simulink model "INS"  (R2018b)
settings: configuration reference "ins_config" (kept outside this file)
values from neighbouring files (symbols this model uses):
  INS_EXPORT = Simulink.Parameter(INS_EXPORT_VALUE)    [ins_model_init.m]
  INS_PARAM = Simulink.Parameter(INS_PARAM_VALUE)    [ins_model_init.m]
undefined symbols (not defined in the file or in its folder): DiscIntNeverNeededParam, INS_CONST, INS_EXPORT_VALUE, Sensor_Meas
libraries: simulink x131, FMT_Model_Lib x48
(part 1 of 6)
settings Model: SimulationMode=accelerator  Creator=jc  LastModifiedBy=zouji
settings ConfigSetRef: SourceLocation=Base Workspace

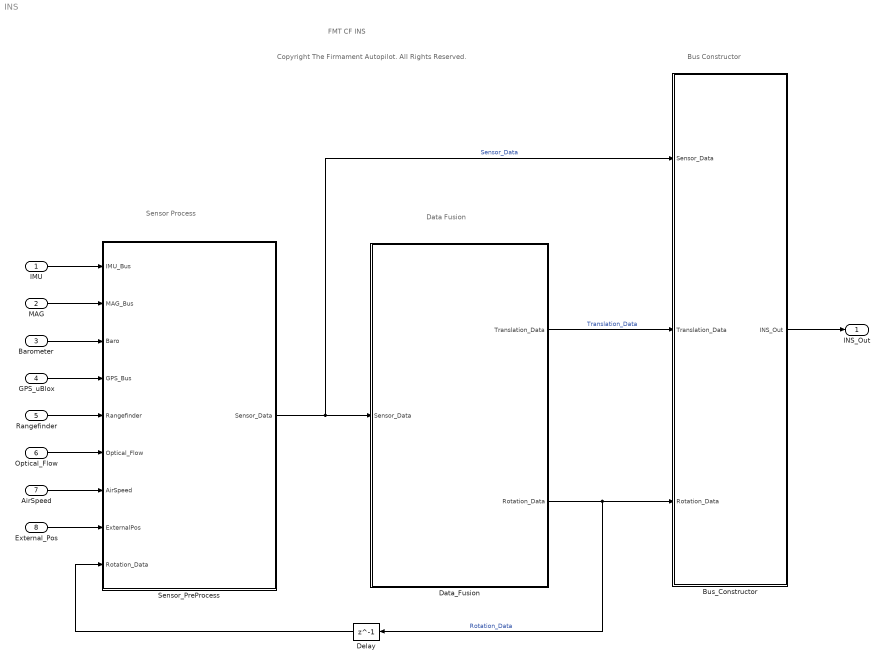
== system INS ==
  note: FMT CF INS
  note: Sensor Process
  note: Data Fusion
  note: Bus Constructor
  note: Copyright The Firmament Autopilot. All Rights Reserved.
  IMU : Inport  OutDataTypeStr=Bus: IMU_Bus  PortDimensions=[1 1]  SampleTime=[INS_CONST.dt,0]  Interpolate=off  BusOutputAsStruct=on
  MAG : Inport  Port=2  OutDataTypeStr=Bus: MAG_Bus  PortDimensions=[1 1]  SampleTime=[INS_CONST.dt,0]  Interpolate=off  BusOutputAsStruct=on
  Barometer : Inport  Port=3  OutDataTypeStr=Bus: Barometer_Bus  PortDimensions=[1 1]  SampleTime=[INS_CONST.dt,0]  Interpolate=off  BusOutputAsStruct=on
  GPS_uBlox : Inport  Port=4  OutDataTypeStr=Bus: GPS_uBlox_Bus  PortDimensions=[1 1]  SampleTime=[INS_CONST.dt,0]  Interpolate=off  BusOutputAsStruct=on
  Rangefinder : Inport  Port=5  OutDataTypeStr=Bus: Rangefinder_Bus  PortDimensions=1  SampleTime=[INS_CONST.dt,0]  Interpolate=off  BusOutputAsStruct=on
  Optical_Flow : Inport  Port=6  OutDataTypeStr=Bus: Optical_Flow_Bus  PortDimensions=[1 1]  SampleTime=[INS_CONST.dt,0]  Interpolate=off  BusOutputAsStruct=on
  AirSpeed : Inport  Port=7  OutDataTypeStr=Bus: AirSpeed_Bus  PortDimensions=[1 1]  SampleTime=[INS_CONST.dt,0]  Interpolate=off  BusOutputAsStruct=on
  External_Pos : Inport  Port=8  OutDataTypeStr=Bus: External_Pos_Bus  PortDimensions=[1 1]  SampleTime=[INS_CONST.dt,0]  Interpolate=off  BusOutputAsStruct=on
  Bus_Constructor : Subsystem  TreatAsAtomicUnit=on
  Data_Fusion : Subsystem  TreatAsAtomicUnit=on
  Delay : Delay  DelayLength=1
  Sensor_PreProcess : Subsystem  TreatAsAtomicUnit=on
  INS_Out : Outport  OutDataTypeStr=Bus: INS_Out_Bus
  wires:
  IMU/1 -> Sensor_PreProcess/1(IMU_Bus)
  MAG/1 -> Sensor_PreProcess/2(MAG_Bus)
  Barometer/1 -> Sensor_PreProcess/3(Baro)
  GPS_uBlox/1 -> Sensor_PreProcess/4(GPS_Bus)
  Rangefinder/1 -> Sensor_PreProcess/5(Rangefinder)
  Bus_Constructor/1(INS_Out) -> INS_Out/1
  Sensor_PreProcess/1(Sensor_Data) -> Bus_Constructor/1(Sensor_Data), Data_Fusion/1(Sensor_Data)  "Sensor_Data"
  Data_Fusion/2(Rotation_Data) -> Delay/1, Bus_Constructor/3(Rotation_Data)  "Rotation_Data"
  Data_Fusion/1(Translation_Data) -> Bus_Constructor/2(Translation_Data)  "Translation_Data"
  Delay/1 -> Sensor_PreProcess/9(Rotation_Data)
  Optical_Flow/1 -> Sensor_PreProcess/6(Optical_Flow)
  AirSpeed/1 -> Sensor_PreProcess/7(AirSpeed)
  External_Pos/1 -> Sensor_PreProcess/8(ExternalPos)

== system INS/Bus_Constructor ==
  Sensor_Data : Inport
  Translation_Data : Inport  Port=2
  Rotation_Data : Inport  Port=3
  Bus Creator : BusCreator  Inputs=29  OutDataTypeStr=Bus: INS_Out_Bus
      settings: InheritFromInputs=off
  Counter : Subsystem  TreatAsAtomicUnit=on
  Rotation_Output : Subsystem  TreatAsAtomicUnit=on
  Status_Output : Subsystem  TreatAsAtomicUnit=on
  Translation_Output : Subsystem  TreatAsAtomicUnit=on
  INS_Out : Outport  OutDataTypeStr=Bus: INS_Out_Bus
  wires:
  Bus Creator/1 -> INS_Out/1
  Counter/1(timestamp_ms) -> Bus Creator/1  "timestamp"
  Rotation_Output/2(theta) -> Bus Creator/3  "theta"
  Rotation_Output/1(phi) -> Bus Creator/2  "phi"
  Rotation_Output/4(att_quat) -> Bus Creator/5  "quat"
  Rotation_Output/3(psi) -> Bus Creator/4  "psi"
  Rotation_Output/5(p) -> Bus Creator/6  "p"
  Rotation_Output/6(q) -> Bus Creator/7  "q"
  Rotation_Output/7(r) -> Bus Creator/8  "r"
  Rotation_Output/8(ax) -> Bus Creator/9  "ax"
  Rotation_Output/9(ay) -> Bus Creator/10  "ay"
  Rotation_Output/10(az) -> Bus Creator/11  "az"
  Translation_Output/1(velN) -> Bus Creator/12  "vn"
  Translation_Output/2(velE) -> Bus Creator/13  "ve"
  Translation_Output/3(velD) -> Bus Creator/14  "vd"
  Status_Output/1(flags) -> Bus Creator/28  "flag"
  Status_Output/2(status) -> Bus Creator/29  "status"
  Translation_Output/13(x_R_m) -> Bus Creator/24  "x_R"
  Translation_Output/14(y_R_m) -> Bus Creator/25  "y_R"
  Translation_Output/15(h_R_m) -> Bus Creator/26  "h_R"
  Translation_Output/16(h_AGL_m) -> Bus Creator/27  "h_AGL"
  Translation_Data/1 -> Status_Output/1(Translation_Data), Translation_Output/1(Translation_Data), Rotation_Output/2(Translation_Data)
  Rotation_Data/1 -> Status_Output/2(Rotation_Data), Rotation_Output/1(Rotation_Data)
  Sensor_Data/1 -> Status_Output/3(Sensor_Data)
  Translation_Output/5(latitude) -> Bus Creator/16  "lat"
  Translation_Output/6(longitude) -> Bus Creator/17  "lon"
  Translation_Output/7(altitude) -> Bus Creator/18  "alt"
  Translation_Output/8(latitude_0) -> Bus Creator/19  "lat_0"
  Translation_Output/9(lontitude_0) -> Bus Creator/20  "lon_0"
  Translation_Output/10(altitude_0) -> Bus Creator/21  "alt_0"
  Translation_Output/4(airspeed) -> Bus Creator/15  "airspeed"
  Translation_Output/11(dx_dlat) -> Bus Creator/22  "dx_dlat"
  Translation_Output/12(dy_dlon) -> Bus Creator/23  "dy_dlon"

== system INS/Data_Fusion ==
  Sensor_Data : Inport
  Delay : Delay  DelayLength=1
  Rotation_Filter : Subsystem
  Translation_Filter : Subsystem
  Translation_Data : Outport
  Rotation_Data : Outport  Port=2
  wires:
  Rotation_Filter/1(Rotation_Data) -> Translation_Filter/2(Rotation_Data), Rotation_Data/1
  Translation_Filter/1(Translation_Data) -> Delay/1, Translation_Data/1
  Sensor_Data/1 -> Rotation_Filter/1(Sensor_Data), Translation_Filter/1(Sensor_Data)
  Delay/1 -> Rotation_Filter/2(Translation_Data)

== system INS/Sensor_PreProcess ==
  IMU_Bus : Inport  Interpolate=off  BusOutputAsStruct=on
  MAG_Bus : Inport  Port=2  Interpolate=off  BusOutputAsStruct=on
  Baro : Inport  Port=3  Interpolate=off  BusOutputAsStruct=on
  GPS_Bus : Inport  Port=4  Interpolate=off  BusOutputAsStruct=on
  Rangefinder : Inport  Port=5
  Optical_Flow : Inport  Port=6
  AirSpeed : Inport  Port=7
  ExternalPos : Inport  Port=8
  Rotation_Data : Inport  Port=9
  AirSpeed_Process : Subsystem  TreatAsAtomicUnit=on
  Baro_PreProcess : Subsystem  TreatAsAtomicUnit=on
  Bus Creator : BusCreator  Inputs=8
  ExternalPos_Process : Subsystem  TreatAsAtomicUnit=on
  GPS_PreProcess : Subsystem  TreatAsAtomicUnit=on
  IMU_PreProcess : Subsystem  TreatAsAtomicUnit=on
  MAG_PreProcess : Subsystem  TreatAsAtomicUnit=on
  OpticalFlow_PreProcess : Subsystem  TreatAsAtomicUnit=on
  Rangefinder_PreProcess : Subsystem  TreatAsAtomicUnit=on
  Sensor_Data : Outport
  wires:
  IMU_Bus/1 -> OpticalFlow_PreProcess/2(IMU_Data), IMU_PreProcess/1(IMU_Bus)
  GPS_Bus/1 -> GPS_PreProcess/1(GPS_Bus)
  GPS_PreProcess/1(GPS_Data) -> MAG_PreProcess/3(GPS_Data), Bus Creator/3  "GPS_Data"
  MAG_Bus/1 -> MAG_PreProcess/1(MAG_Bus)
  Rotation_Data/1 -> Rangefinder_PreProcess/1(Rotation_Data), MAG_PreProcess/2(Rotation_Data)
  Baro/1 -> Baro_PreProcess/1(Baro)
  IMU_PreProcess/1(IMU_Data) -> Bus Creator/1  "IMU_Data"
  MAG_PreProcess/1(Mag_Data) -> Bus Creator/2  "Mag_Data"
  Baro_PreProcess/1(Baro_Data) -> Bus Creator/4  "Baro_Data"
  Bus Creator/1 -> Sensor_Data/1
  Rangefinder/1 -> Rangefinder_PreProcess/2(Rangefinder_Bus)
  Rangefinder_PreProcess/1(Rangefinder_Data) -> OpticalFlow_PreProcess/1(Rangefinder_Data), Bus Creator/5  "Rangefinder_Data"
  OpticalFlow_PreProcess/1(OpticalFlow_Data) -> Bus Creator/6  "OpticalFlow_Data"
  Optical_Flow/1 -> OpticalFlow_PreProcess/3(OpticalFlow_Bus)
  AirSpeed_Process/1(AirSpeed_Data) -> Bus Creator/7  "AirSpeed_Data"
  AirSpeed/1 -> AirSpeed_Process/1(AirSpeed)
  ExternalPos/1 -> ExternalPos_Process/1(ExternalPos)
  ExternalPos_Process/1(ExternalPos_Data) -> Bus Creator/8  "ExternalPos_Data"

== system INS/Bus_Constructor/Counter ==
  Add : Sum
  Constant : Constant  Value=INS_EXPORT.period  OutDataTypeStr=uint32
  Data Type Conversion : DataTypeConversion  OutDataTypeStr=uint32
  Output : UnitDelay  InitialCondition=0.0  SampleTime=-1
  timestamp_ms : Outport
  wires:
  Add/1 -> Output/1
  Output/1 -> Add/2, Data Type Conversion/1
  Data Type Conversion/1 -> timestamp_ms/1
  Constant/1 -> Add/1

== system INS/Bus_Constructor/Rotation_Output ==
  Rotation_Data : Inport
  Translation_Data : Inport  Port=2
  Bus Selector : BusSelector  OutputSignals=ba_mPs2
  Bus Selector3 : BusSelector  OutputSignals=phi_rad,theta_rad,psi_rad,att_quat,gyr_B_radPs,acc_B_mPs2,M_BO
  Demux3 : Demux  Outputs=3
  Demux4 : Demux  Outputs=3
  Multiply : Product  Multiplication=Matrix(*)
  Signal Copy : SignalConversion  OverrideOpt=off
  Sum : Sum  Inputs=|+-
  phi : Outport
  theta : Outport  Port=2
  psi : Outport  Port=3
  att_quat : Outport  Port=4
  p : Outport  Port=5
  q : Outport  Port=6
  r : Outport  Port=7
  ax : Outport  Port=8
  ay : Outport  Port=9
  az : Outport  Port=10
  wires:
  Bus Selector/1 -> Multiply/2  "<ba_mPs2>"
  Demux4/1 -> ax/1  "acc_x"
  Demux3/3 -> r/1  "gyr_z"
  Demux3/2 -> q/1  "gyr_y"
  Demux3/1 -> p/1  "gyr_x"
  Bus Selector3/5 -> Demux3/1  "<gyr_B_radPs>"
  Sum/1 -> Demux4/1
  Bus Selector3/1 -> phi/1  "<phi_rad>"
  Bus Selector3/6 -> Sum/1  "<acc_B_mPs2>"
  Demux4/3 -> az/1  "acc_z"
  Demux4/2 -> ay/1  "acc_y"
  Bus Selector3/2 -> theta/1  "<theta_rad>"
  Bus Selector3/3 -> psi/1  "<psi_rad>"
  Bus Selector3/7 -> Multiply/1  "<M_BO>"
  Multiply/1 -> Sum/2
  Bus Selector3/4 -> att_quat/1  "<att_quat>"
  Rotation_Data/1 -> Signal Copy/1
  Signal Copy/1 -> Bus Selector3/1
  Translation_Data/1 -> Bus Selector/1

== system INS/Bus_Constructor/Status_Output ==
  Translation_Data : Inport
  Rotation_Data : Inport  Port=2
  Sensor_Data : Inport  Port=3
  INS_Flag : Subsystem
  INS_Quality : Subsystem
  Sensor_Status : Subsystem
  flags : Outport
  status : Outport  Port=2
  wires:
  INS_Flag/1(flags) -> flags/1
  Sensor_Status/1(status) -> status/1
  INS_Quality/1(ins_valid) -> INS_Flag/1(INS_Valid)
  Rotation_Data/1 -> INS_Flag/3(Rotation_Data)
  Sensor_Data/1 -> Sensor_Status/1(Sensor_Data), INS_Flag/2(Sensor_Data), INS_Quality/2(Sensor_Data)
  Translation_Data/1 -> INS_Quality/1(Translation_Data)

== system INS/Bus_Constructor/Translation_Output ==
  Translation_Data : Inport
  Bus Selector4 : BusSelector  OutputSignals=vn_mPs,ve_mPs,vd_mPs,TAS_mPs,lat_rad,lon_rad,h_m,lat_0_rad,lon_0_rad,h_0_m,dx_dlat,dy_dlon,x_R_m,y_R_m,h_R_m,h_gnd_m
  Signal Copy : SignalConversion  OverrideOpt=off
  velN : Outport
  velE : Outport  Port=2
  velD : Outport  Port=3
  airspeed : Outport  Port=4
  latitude : Outport  Port=5
  longitude : Outport  Port=6
  altitude : Outport  Port=7
  latitude_0 : Outport  Port=8
  lontitude_0 : Outport  Port=9
  altitude_0 : Outport  Port=10
  dx_dlat : Outport  Port=11
  dy_dlon : Outport  Port=12
  x_R_m : Outport  Port=13
  y_R_m : Outport  Port=14
  h_R_m : Outport  Port=15
  h_AGL_m : Outport  Port=16
  wires:
  Bus Selector4/5 -> latitude/1  "<lat_rad>"
  Bus Selector4/6 -> longitude/1  "<lon_rad>"
  Bus Selector4/2 -> velE/1  "<ve_mPs>"
  Bus Selector4/3 -> velD/1  "<vd_mPs>"
  Bus Selector4/7 -> altitude/1  "<h_m>"
  Bus Selector4/1 -> velN/1  "<vn_mPs>"
  Bus Selector4/16 -> h_AGL_m/1  "<h_gnd_m>"
  Bus Selector4/15 -> h_R_m/1  "<h_R_m>"
  Bus Selector4/13 -> x_R_m/1  "<x_R_m>"
  Bus Selector4/14 -> y_R_m/1  "<y_R_m>"
  Translation_Data/1 -> Signal Copy/1
  Bus Selector4/8 -> latitude_0/1  "<lat_0_rad>"
  Bus Selector4/9 -> lontitude_0/1  "<lon_0_rad>"
  Bus Selector4/10 -> altitude_0/1  "<h_0_m>"
  Bus Selector4/11 -> dx_dlat/1  "<dx_dlat>"
  Bus Selector4/12 -> dy_dlon/1  "<dy_dlon>"
  Signal Copy/1 -> Bus Selector4/1
  Bus Selector4/4 -> airspeed/1  "<TAS_mPs>"

== system INS/Data_Fusion/Rotation_Filter ==
  Sensor_Data : Inport
  Translation_Data : Inport  Port=2
  AHRS : Subsystem  TreatAsAtomicUnit=on
  RF_Data_PreProcess : Subsystem  TreatAsAtomicUnit=on
  Rotation_Data : Outport
  wires:
  Sensor_Data/1 -> AHRS/2(Sensor_Data), RF_Data_PreProcess/1(Sensor_Data)
  AHRS/1(Rotation_Data) -> Rotation_Data/1
  RF_Data_PreProcess/1(RF_Data) -> AHRS/1(RF_Data)  "RF_Data"
  Translation_Data/1 -> AHRS/3(Translation_Data)

== system INS/Data_Fusion/Translation_Filter ==
  Sensor_Data : Inport
  Rotation_Data : Inport  Port=2
  CF : Subsystem  TreatAsAtomicUnit=on
  Delay : Delay  DelayLength=1
  TF_Data_PreProcess : Subsystem  TreatAsAtomicUnit=on
  Translation_Data : Outport
  wires:
  CF/1(Translation_Data) -> Delay/1, Translation_Data/1
  TF_Data_PreProcess/1(TF_Data) -> CF/1(TF_Data)  "TF_Data"
  Sensor_Data/1 -> TF_Data_PreProcess/1(Sensor_Data)
  Delay/1 -> TF_Data_PreProcess/3(Translation_Data)
  Rotation_Data/1 -> TF_Data_PreProcess/2(Rotation_Data), CF/2(Rotation_Data)

== system INS/Sensor_PreProcess/AirSpeed_Process ==
  AirSpeed : Inport
  Bus Creator : BusCreator  Inputs=3
  Bus Selector : BusSelector  OutputSignals=timestamp,diff_pressure
  Calculate_IAS : Subsystem
  Saturation1 : Saturate  UpperLimit=999  LowerLimit=0.1
  Sensor_Valid : Subsystem  mask{max_pressure=1e4, min_pressure=-1e4, max_temp=80, min_temp=-20, timeout=200}
      mask prompts: max_pressure "Max pressure (Pa)"; min_pressure "Min pressure (Pa)"; max_temp "Max temprature (deg)"; min_temp "Min temprature (deg)"; timeout "Timeout (ms)"
  AirSpeed_Data : Outport
  wires:
  Bus Creator/1 -> AirSpeed_Data/1
  AirSpeed/1 -> Bus Selector/1, Sensor_Valid/1(Airspeed)
  Bus Selector/1 -> Bus Creator/1  "<timestamp>"
  Bus Selector/2 -> Calculate_IAS/1(diff_pressure)  "<diff_pressure>"
  Calculate_IAS/1(IAS) -> Saturation1/1
  Saturation1/1 -> Bus Creator/2  "IAS"
  Sensor_Valid/1(valid) -> Bus Creator/3  "valid"

== system INS/Sensor_PreProcess/Baro_PreProcess ==
  Baro : Inport
  Bus Creator : BusCreator  Inputs=5
  Bus Selector1 : BusSelector  OutputSignals=pressure
  Bus Selector2 : BusSelector  OutputSignals=temperature,timestamp
  Pressure_Height : Subsystem
  Relative_Height : Subsystem
  Sensor_Valid : Subsystem  mask{max_pressure=110e3, min_pressure=30e3, max_temp=70, min_temp=-20, timeout=200}
      mask prompts: max_pressure "Max pressure (Pa)"; min_pressure "Min pressure (Pa)"; max_temp "Max temprature (deg)"; min_temp "Min temprature (deg)"; timeout "Timeout (ms)"
  Baro_Data : Outport
  wires:
  Bus Selector1/1 -> Pressure_Height/1(pressure_Pa)  "<pressure>"
  Baro/1 -> Bus Selector2/1, Bus Selector1/1, Sensor_Valid/1(Baro), Relative_Height/1(Baro)
  Bus Creator/1 -> Baro_Data/1
  Bus Selector2/1 -> Bus Creator/4  "<temperature>"
  Bus Selector2/2 -> Bus Creator/5  "<timestamp>"
  Pressure_Height/1(h_FL_m) -> Relative_Height/3(h_FL_m), Bus Creator/3  "h_FL_m"
  Sensor_Valid/1(valid) -> Relative_Height/2(data_valid)
  Relative_Height/2(baro_valid) -> Bus Creator/2  "baro_valid"
  Relative_Height/1(h_R_m) -> Bus Creator/1  "h_R_m"

== system INS/Sensor_PreProcess/ExternalPos_Process ==
  ExternalPos : Inport
  Bus Creator : BusCreator  Inputs=11
  Bus Selector : BusSelector  OutputSignals=timestamp,field_valid
  Bus_Selector : Subsystem
  Sensor_Valid : Subsystem  mask{timeout=200}
      mask prompts: timeout "Timeout (ms)"
  Signal Copy : SignalConversion  OverrideOpt=off
  ExternalPos_Data : Outport
  wires:
  Bus Creator/1 -> ExternalPos_Data/1
  ExternalPos/1 -> Bus_Selector/1(ExternalPos), Bus Selector/1
  Bus Selector/1 -> Signal Copy/1, Sensor_Valid/1(timestamp)  "<timestamp>"
  Signal Copy/1 -> Bus Creator/1  "timestamp"
  Sensor_Valid/1(pos_valid) -> Bus Creator/2  "pos_valid"
  Sensor_Valid/2(height_valid) -> Bus Creator/3  "height_valid"
  Sensor_Valid/3(att_valid) -> Bus Creator/4  "att_valid"
  Sensor_Valid/4(heading_valid) -> Bus Creator/5  "heading_valid"
  Bus_Selector/1(x) -> Bus Creator/6  "x"
  Bus_Selector/2(y) -> Bus Creator/7  "y"
  Bus_Selector/3(h) -> Bus Creator/8  "h"
  Bus_Selector/4(phi) -> Bus Creator/9  "phi"
  Bus_Selector/5(theta) -> Bus Creator/10  "theta"
  Bus_Selector/6(psi) -> Bus Creator/11  "psi"
  Bus Selector/2 -> Sensor_Valid/2(field_valid)  "<field_valid>"

== system INS/Sensor_PreProcess/GPS_PreProcess ==
  GPS_Bus : Inport  Interpolate=off  BusOutputAsStruct=on
  Bus Creator1 : BusCreator  Inputs=20
  Compare To Constant : simulink/Logic and Bit Operations/Compare To Constant  relop=>  const=0  OutDataTypeStr=boolean
  Compare To Constant1 : simulink/Logic and Bit Operations/Compare To Constant  relop===  const=2  OutDataTypeStr=boolean
  Data_Scalling : Subsystem
  Status_Quality : Subsystem
  WGS84_Model : Subsystem
  GPS_Data : Outport
  wires:
  Compare To Constant1/1 -> Bus Creator1/1  "GPS_valid"
  WGS84_Model/5(dz_dh) -> Bus Creator1/10  "dz_dh"
  GPS_Bus/1 -> Data_Scalling/1(GPS_Bus), Status_Quality/1(GPS_Bus)
  Compare To Constant/1 -> WGS84_Model/Trigger
  Bus Creator1/1 -> GPS_Data/1
  Status_Quality/1(gps_status) -> Compare To Constant/1, Compare To Constant1/1
  WGS84_Model/2(lat_0_rad) -> Bus Creator1/7  "lat_0_rad"
  WGS84_Model/3(dx_dlat) -> Bus Creator1/8  "dx_dlat"
  WGS84_Model/4(dy_dlon) -> Bus Creator1/9  "dy_dlon"
  Status_Quality/2(spd_quality) -> Bus Creator1/2  "spd_quality"
  Status_Quality/3(hor_pos_quality) -> Bus Creator1/3  "pos_quality"
  Data_Scalling/2(lon_O_rad) -> WGS84_Model/2(lon_rad), Bus Creator1/12  "lon_rad"
  Data_Scalling/3(height_O_m) -> WGS84_Model/3(alt_m), Bus Creator1/13  "height_m"
  Data_Scalling/1(lat_O_rad) -> Bus Creator1/11, WGS84_Model/1(lat_rad)  "lat_rad"
  Data_Scalling/4(vn_O_mPs) -> Bus Creator1/14  "vn_mPs"
  Data_Scalling/5(ve_O_mPs) -> Bus Creator1/15  "ve_mPs"
  Data_Scalling/6(vd_O_mPs) -> Bus Creator1/16  "vd_mPs"
  Data_Scalling/8(numSV) -> Bus Creator1/18  "numSV"
  Data_Scalling/10(timestamp_ms) -> Bus Creator1/20  "timestamp_ms"
  WGS84_Model/1(lon_0_rad) -> Bus Creator1/6  "lon_0_rad"
  Status_Quality/4(ver_pos_quality) -> Bus Creator1/4  "alt_quality"
  Data_Scalling/9(fixType) -> Bus Creator1/19  "fixType"
  Data_Scalling/7(heading_rad) -> Bus Creator1/17  "heading_rad"
  Status_Quality/5(heading_valid) -> Bus Creator1/5  "heading_valid"

== system INS/Sensor_PreProcess/IMU_PreProcess ==
  IMU_Bus : Inport
  Bus Creator : BusCreator  Inputs=3
  Data_Select : Subsystem
  Sensor_Valid : Subsystem  mask{gyr_min=-2200*pi/180, gyr_max=2200*pi/180, acc_min=-10*INS_CONST.g, acc_max=10*INS_CONST.g, timeout=100}
      mask prompts: gyr_min "Gyro min (rad/s)"; gyr_max "Gyro max (rad/s)"; acc_min "Accel min (m/s2)"; acc_max "Accel max (m/s2)"; timeout "Timeout (ms)"
  IMU_Data : Outport
  wires:
  Bus Creator/1 -> IMU_Data/1
  Sensor_Valid/1(valid) -> Bus Creator/3  "IMU_valid"
  Data_Select/3(timestamp_ms) -> Sensor_Valid/3(timestamp_ms)
  Data_Select/2(acc_B_mPs2) -> Bus Creator/2, Sensor_Valid/2(acc_B_mPs2)  "acc_B_mPs2"
  Data_Select/1(gyr_B_radPs) -> Bus Creator/1, Sensor_Valid/1(gyr_B_radPs)  "gyr_B_radPs"
  IMU_Bus/1 -> Data_Select/1(IMU_Bus)

== system INS/Sensor_PreProcess/MAG_PreProcess ==
  MAG_Bus : Inport
  Rotation_Data : Inport  Port=2
  GPS_Data : Inport  Port=3
  Bus Creator : BusCreator  Inputs=3
  Bus Selector4 : BusSelector  OutputSignals=M_OB
  Bus_Select : Subsystem
  Gauss_to_uT : Gain  Gain=100
  Mag_Data_Process : Subsystem
  Sensor_Valid : Subsystem  mask{mag_min=-30000, mag_max=30000, timeout=1000}
      mask prompts: mag_min "Mag min (gauss)"; mag_max "Mag max (gauss)"; timeout "Timeout (ms)"
  Mag_Data : Outport
  wires:
  Rotation_Data/1 -> Bus Selector4/1
  Bus Selector4/1 -> Mag_Data_Process/3(DCM_OB)  "<M_OB>"
  Gauss_to_uT/1 -> Mag_Data_Process/1(mag_B_uT)
  MAG_Bus/1 -> Bus_Select/1(MAG_Bus)
  Mag_Data_Process/1(mag_normalized_B) -> Bus Creator/1  "mag_norm_B"
  GPS_Data/1 -> Mag_Data_Process/4(GPS_Data)
  Mag_Data_Process/2(mag_quality) -> Bus Creator/2  "mag_quality"
  Bus Creator/1 -> Mag_Data/1
  Bus_Select/1(mag_B_gauss) -> Gauss_to_uT/1, Sensor_Valid/1(mag_B_gauss)
  Bus_Select/2(timestamp_ms) -> Sensor_Valid/2(timestamp_ms)
  Sensor_Valid/1(valid) -> Bus Creator/3, Mag_Data_Process/2(mag_valid)  "mag_valid"

== system INS/Sensor_PreProcess/OpticalFlow_PreProcess ==
  Rangefinder_Data : Inport
  IMU_Data : Inport  Port=2
  OpticalFlow_Bus : Inport  Port=3
  Bus Creator : BusCreator  Inputs=4
  Bus Selector : BusSelector  OutputSignals=timestamp
  Height_Compensation : Subsystem
  Sensor_Valid : Subsystem  mask{max_vel=20, min_vel=-20, q_high=90, q_low=50, timeout=100}
      mask prompts: max_vel "Max Velocity (m/s)"; min_vel "Min Velocity (m/s)"; q_high "Quality Threshold High"; q_low "Quality Threshold Low"; timeout "Timeout (ms)"
  OpticalFlow_Data : Outport
  wires:
  Bus Creator/1 -> OpticalFlow_Data/1
  Sensor_Valid/1(valid) -> Bus Creator/2  "valid"
  OpticalFlow_Bus/1 -> Height_Compensation/1(OpticalFlow_Bus), Bus Selector/1, Sensor_Valid/1(OpticalFlow_Bus)
  Rangefinder_Data/1 -> Sensor_Valid/2(Rangefinder_Data), Height_Compensation/3(Rangefinder_Data)
  Height_Compensation/1(vx_B_mPs) -> Bus Creator/3  "vx"
  Height_Compensation/2(vy_B_mPs) -> Bus Creator/4  "vy"
  Bus Selector/1 -> Bus Creator/1  "<timestamp>"
  IMU_Data/1 -> Height_Compensation/2(IMU_Data)

== system INS/Sensor_PreProcess/Rangefinder_PreProcess ==
  Rotation_Data : Inport
  Rangefinder_Bus : Inport  Port=2
  Bus Creator : BusCreator  Inputs=4
  Bus Selector : BusSelector  OutputSignals=timestamp
  Sensor_Valid : Subsystem  mask{max_alt=4, min_alt=0, timeout=100}
      mask prompts: max_alt "Max Altitude (m)"; min_alt "Min Altitude (m)"; timeout "Timeout (ms)"
  Subsystem : Subsystem
  Tilt_Compensation : Subsystem
  Rangefinder_Data : Outport
  wires:
  Rangefinder_Bus/1 -> Bus Selector/1, Sensor_Valid/1(Rangefinder_Bus), Tilt_Compensation/1(Rangefinder_Bus)
  Sensor_Valid/1(valid) -> Subsystem/1(in)
  Bus Creator/1 -> Rangefinder_Data/1
  Rotation_Data/1 -> Tilt_Compensation/2(Rotation_Data)
  Tilt_Compensation/2(distance) -> Bus Creator/4  "distance"
  Tilt_Compensation/1(raw_distance) -> Bus Creator/3  "raw_distance"
  Bus Selector/1 -> Bus Creator/1  "<timestamp>"
  Subsystem/1(out) -> Bus Creator/2  "valid"

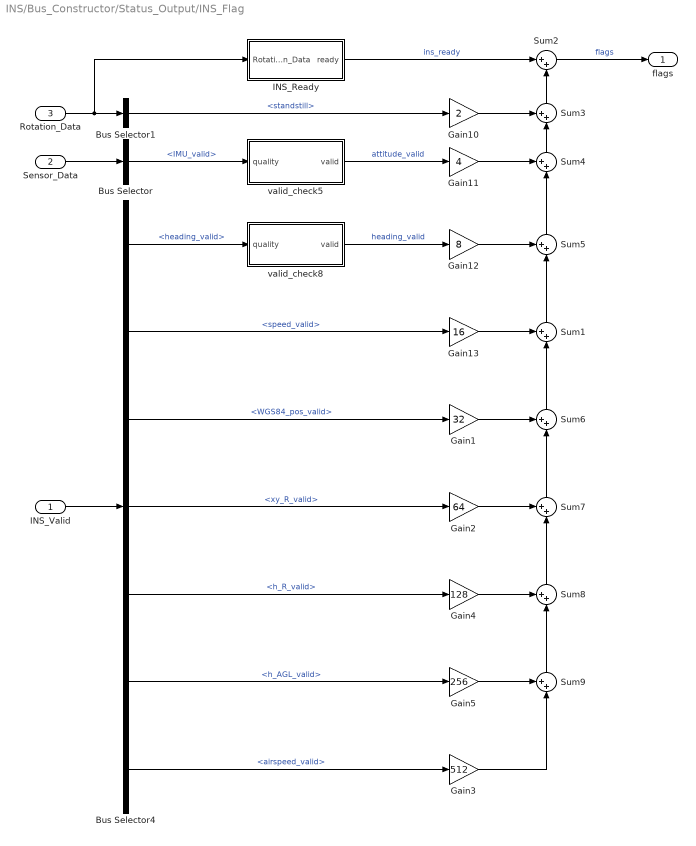
== system INS/Bus_Constructor/Status_Output/INS_Flag ==
  INS_Valid : Inport
  Sensor_Data : Inport  Port=2
  Rotation_Data : Inport  Port=3
  Bus Selector : BusSelector  OutputSignals=IMU_Data.IMU_valid
  Bus Selector1 : BusSelector  OutputSignals=standstill
  Bus Selector4 : BusSelector  OutputSignals=heading_valid,speed_valid,WGS84_pos_valid,xy_R_valid,h_R_valid,h_AGL_valid,airspeed_valid
  Gain1 : Gain  Gain=32  OutDataTypeStr=uint32
  Gain10 : Gain  Gain=2  OutDataTypeStr=uint32
  Gain11 : Gain  Gain=4  OutDataTypeStr=uint32
  Gain12 : Gain  Gain=8  OutDataTypeStr=uint32
  Gain13 : Gain  Gain=16  OutDataTypeStr=uint32
  Gain2 : Gain  Gain=64  OutDataTypeStr=uint32
  Gain3 : Gain  Gain=512  OutDataTypeStr=uint32
  Gain4 : Gain  Gain=128  OutDataTypeStr=uint32
  Gain5 : Gain  Gain=256  OutDataTypeStr=uint32
  INS_Ready : Subsystem
  Sum{1,3..9} (8 alike) : Sum  Inputs=++|
  Sum2 : Sum  Inputs=|++
  valid_check5 : Subsystem  mask{time_out=100}
      mask prompts: time_out "timeout in ms"
  valid_check8 : Subsystem  mask{time_out=1000}
      mask prompts: time_out "timeout in ms"
  flags : Outport
  wires:
  Bus Selector/1 -> valid_check5/1(quality)  "<IMU_valid>"
  Gain1/1 -> Sum6/1
  Sum1/1 -> Sum5/2
  Gain13/1 -> Sum1/1
  valid_check5/1(valid) -> Gain11/1  "attitude_valid"
  Bus Selector4/3 -> Gain1/1  "<WGS84_pos_valid>"
  Bus Selector4/2 -> Gain13/1  "<speed_valid>"
  Bus Selector4/1 -> valid_check8/1(quality)  "<heading_valid>"
  INS_Valid/1 -> Bus Selector4/1
  Sum2/1 -> flags/1  "flags"
  Sum5/1 -> Sum4/2
  INS_Ready/1(ready) -> Sum2/1  "ins_ready"
  Gain11/1 -> Sum4/1
  Gain12/1 -> Sum5/1
  Sum3/1 -> Sum2/2
  Sum4/1 -> Sum3/2
  Sensor_Data/1 -> Bus Selector/1
  Gain10/1 -> Sum3/1
  Sum6/1 -> Sum1/2
  Sum7/1 -> Sum6/2
  Rotation_Data/1 -> INS_Ready/1(Rotation_Data), Bus Selector1/1
  Gain2/1 -> Sum7/1
  Sum8/1 -> Sum7/2
  Gain4/1 -> Sum8/1
  Bus Selector4/4 -> Gain2/1  "<xy_R_valid>"
  Bus Selector4/5 -> Gain4/1  "<h_R_valid>"
  Bus Selector4/6 -> Gain5/1  "<h_AGL_valid>"
  valid_check8/1(valid) -> Gain12/1  "heading_valid"
  Bus Selector4/7 -> Gain3/1  "<airspeed_valid>"
  Sum9/1 -> Sum8/2
  Gain5/1 -> Sum9/1
  Gain3/1 -> Sum9/2
  Bus Selector1/1 -> Gain10/1  "<standstill>"

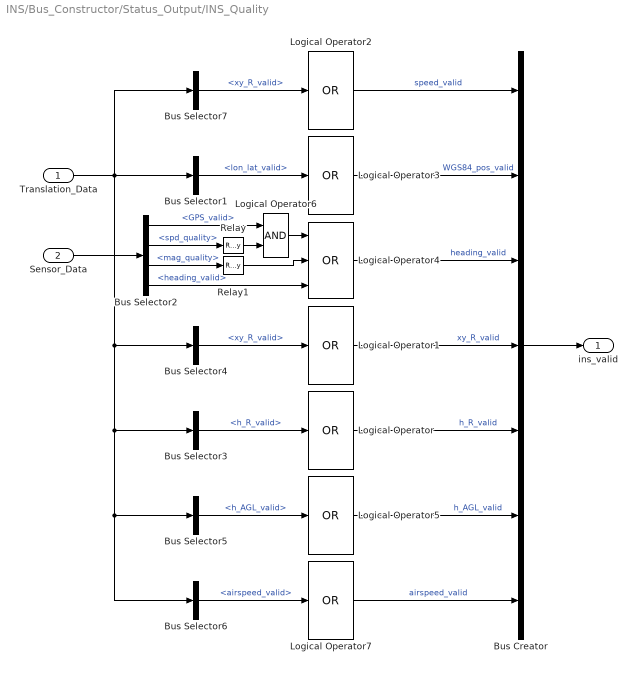
== system INS/Bus_Constructor/Status_Output/INS_Quality ==
  Translation_Data : Inport
  Sensor_Data : Inport  Port=2
  Bus Creator : BusCreator  Inputs=7
  Bus Selector1 : BusSelector  OutputSignals=sensor_valid.lon_lat_valid
  Bus Selector2 : BusSelector  OutputSignals=GPS_Data.GPS_valid,GPS_Data.spd_quality,Mag_Data.mag_quality,ExternalPos_Data.heading_valid
  Bus Selector3 : BusSelector  OutputSignals=sensor_valid.h_R_valid
  Bus Selector4 : BusSelector  OutputSignals=sensor_valid.xy_R_valid
  Bus Selector5 : BusSelector  OutputSignals=sensor_valid.h_AGL_valid
  Bus Selector6 : BusSelector  OutputSignals=sensor_valid.airspeed_valid
  Bus Selector7 : BusSelector  OutputSignals=sensor_valid.xy_R_valid
  Logical Operator{,1..3,5,7} (6 alike) : Logic  Operator=OR  Inputs=1  AllPortsSameDT=off  OutDataTypeStr=boolean
  Logical Operator4 : Logic  Operator=OR  Inputs=3  AllPortsSameDT=off  OutDataTypeStr=boolean
  Logical Operator6 : Logic  AllPortsSameDT=off  OutDataTypeStr=boolean
  Relay : Relay  OnSwitchValue=0.2  OffSwitchValue=0.1
  Relay1 : Relay  OnSwitchValue=0.3  OffSwitchValue=0.2  OutDataTypeStr=boolean
  ins_valid : Outport
  wires:
  Bus Creator/1 -> ins_valid/1
  Logical Operator4/1 -> Bus Creator/3  "heading_valid"
  Sensor_Data/1 -> Bus Selector2/1
  Bus Selector2/3 -> Relay1/1  "<mag_quality>"
  Bus Selector7/1 -> Logical Operator2/1  "<xy_R_valid>"
  Logical Operator3/1 -> Bus Creator/2  "WGS84_pos_valid"
  Logical Operator2/1 -> Bus Creator/1  "speed_valid"
  Logical Operator1/1 -> Bus Creator/4  "xy_R_valid"
  Logical Operator/1 -> Bus Creator/5  "h_R_valid"
  Bus Selector5/1 -> Logical Operator5/1  "<h_AGL_valid>"
  Translation_Data/1 -> Bus Selector6/1, Bus Selector5/1, Bus Selector3/1, Bus Selector4/1, Bus Selector1/1, Bus Selector7/1
  Relay1/1 -> Logical Operator4/2
  Bus Selector1/1 -> Logical Operator3/1  "<lon_lat_valid>"
  Bus Selector4/1 -> Logical Operator1/1  "<xy_R_valid>"
  Bus Selector3/1 -> Logical Operator/1  "<h_R_valid>"
  Logical Operator5/1 -> Bus Creator/6  "h_AGL_valid"
  Bus Selector2/2 -> Relay/1  "<spd_quality>"
  Bus Selector2/1 -> Logical Operator6/1  "<GPS_valid>"
  Relay/1 -> Logical Operator6/2
  Logical Operator6/1 -> Logical Operator4/1
  Bus Selector2/4 -> Logical Operator4/3  "<heading_valid>"
  Bus Selector6/1 -> Logical Operator7/1  "<airspeed_valid>"
  Logical Operator7/1 -> Bus Creator/7  "airspeed_valid"

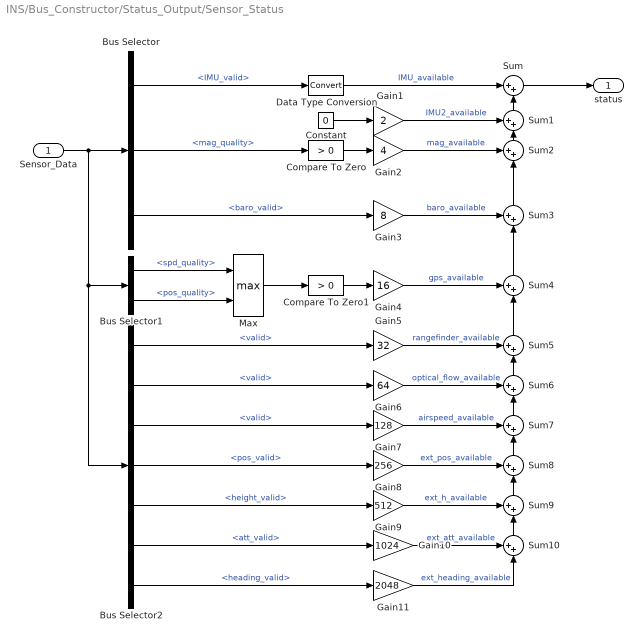
== system INS/Bus_Constructor/Status_Output/Sensor_Status ==
  Sensor_Data : Inport
  Bus Selector : BusSelector  OutputSignals=IMU_Data.IMU_valid,Mag_Data.mag_quality,Baro_Data.baro_valid
  Bus Selector1 : BusSelector  OutputSignals=GPS_Data.spd_quality,GPS_Data.pos_quality
  Bus Selector2 : BusSelector  OutputSignals=Rangefinder_Data.valid,OpticalFlow_Data.valid,AirSpeed_Data.valid,ExternalPos_Data.pos_valid,ExternalPos_Data.height_valid,ExternalPos_Data.att_valid,ExternalPos_Data.heading_valid
  Compare To Zero : simulink/Logic and Bit Operations/Compare To Zero  relop=>  OutDataTypeStr=boolean
  Compare To Zero1 : simulink/Logic and Bit Operations/Compare To Zero  relop=>  OutDataTypeStr=boolean
  Constant : Constant  Value=0  OutDataTypeStr=Inherit: Inherit via back propagation
  Data Type Conversion : DataTypeConversion
  Gain1 : Gain  Gain=2  OutDataTypeStr=uint32
  Gain10 : Gain  Gain=1024  OutDataTypeStr=uint32
  Gain11 : Gain  Gain=2048  OutDataTypeStr=uint32
  Gain2 : Gain  Gain=4  OutDataTypeStr=uint32
  Gain3 : Gain  Gain=8  OutDataTypeStr=uint32
  Gain4 : Gain  Gain=16  OutDataTypeStr=uint32
  Gain5 : Gain  Gain=32  OutDataTypeStr=uint32
  Gain6 : Gain  Gain=64  OutDataTypeStr=uint32
  Gain7 : Gain  Gain=128  OutDataTypeStr=uint32
  Gain8 : Gain  Gain=256  OutDataTypeStr=uint32
  Gain9 : Gain  Gain=512  OutDataTypeStr=uint32
  Max : MinMax  Function=max  Inputs=2
  Sum : Sum  Inputs=|++
  Sum{1..10} (10 alike) : Sum  Inputs=++|
  status : Outport
  wires:
  Max/1 -> Compare To Zero1/1
  Compare To Zero1/1 -> Gain4/1
  Bus Selector1/2 -> Max/2  "<pos_quality>"
  Bus Selector1/1 -> Max/1  "<spd_quality>"
  Sum4/1 -> Sum3/2
  Gain3/1 -> Sum3/1  "baro_available"
  Sum3/1 -> Sum2/2
  Gain2/1 -> Sum2/1  "mag_available"
  Compare To Zero/1 -> Gain2/1
  Sum2/1 -> Sum1/2
  Bus Selector/3 -> Gain3/1  "<baro_valid>"
  Bus Selector/2 -> Compare To Zero/1  "<mag_quality>"
  Sensor_Data/1 -> Bus Selector/1, Bus Selector2/1, Bus Selector1/1
  Sum/1 -> status/1
  Data Type Conversion/1 -> Sum/1  "IMU_available"
  Bus Selector/1 -> Data Type Conversion/1  "<IMU_valid>"
  Constant/1 -> Gain1/1
  Sum1/1 -> Sum/2
  Gain1/1 -> Sum1/1  "IMU2_available"
  Bus Selector2/1 -> Gain5/1  "<valid>"
  Gain4/1 -> Sum4/1  "gps_available"
  Gain5/1 -> Sum5/1  "rangefinder_available"
  Bus Selector2/2 -> Gain6/1  "<valid>"
  Sum5/1 -> Sum4/2
  Gain6/1 -> Sum6/1  "optical_flow_available"
  Sum6/1 -> Sum5/2
  Bus Selector2/3 -> Gain7/1  "<valid>"
  Bus Selector2/4 -> Gain8/1  "<pos_valid>"
  Bus Selector2/5 -> Gain9/1  "<height_valid>"
  Bus Selector2/6 -> Gain10/1  "<att_valid>"
  Bus Selector2/7 -> Gain11/1  "<heading_valid>"
  Sum7/1 -> Sum6/2
  Gain7/1 -> Sum7/1  "airspeed_available"
  Sum8/1 -> Sum7/2
  Gain8/1 -> Sum8/1  "ext_pos_available"
  Sum9/1 -> Sum8/2
  Gain9/1 -> Sum9/1  "ext_h_available"
  Sum10/1 -> Sum9/2
  Gain10/1 -> Sum10/1  "ext_att_available"
  Gain11/1 -> Sum10/2  "ext_heading_available"

== system INS/Data_Fusion/Rotation_Filter/AHRS ==
  RF_Data : Inport
  Sensor_Data : Inport  Port=2
  Translation_Data : Inport  Port=3
  Bus_Constructor : Subsystem  TreatAsAtomicUnit=on
  Correct : Subsystem  TreatAsAtomicUnit=on
  Delay1 : Delay  DelayLength=1
  Delay2 : Delay  DelayLength=1
  Update : Subsystem  TreatAsAtomicUnit=on
  Rotation_Data : Outport
  wires:
  Correct/1(att_B_correction) -> Delay1/1
  Correct/2(bias_g_B_correction) -> Delay2/1
  Sensor_Data/1 -> Bus_Constructor/5(Sensor_Data), Update/4(Sensor_Data), Correct/3(Sensor_Data)
  Update/1(att_quat) -> Bus_Constructor/2(att_quat)
  Update/2(DCM_OB) -> Bus_Constructor/3(DCM_OB)
  Update/3(bias_g) -> Bus_Constructor/4(bias_g)
  RF_Data/1 -> Correct/4(RF_Data), Update/3(RF_Data), Bus_Constructor/1(RF_Data)
  Bus_Constructor/1(Rotation_Data) -> Correct/1(Rotation_Data), Rotation_Data/1
  Delay1/1 -> Update/1(att_B_correction)
  Delay2/1 -> Update/2(bias_g_correction)
  Translation_Data/1 -> Correct/2(Translation_Data)

== system INS/Data_Fusion/Rotation_Filter/RF_Data_PreProcess ==
  Sensor_Data : Inport
  Attitude_Reset : Subsystem
  Bus Creator : BusCreator  Inputs=7
  Bus Selector2 : BusSelector  OutputSignals=IMU_Data
  Initial_Attitude : Subsystem
  Sensor_Select : Subsystem
  Standstill : Subsystem
  RF_Data : Outport
  wires:
  Bus Selector2/1 -> Standstill/1(IMU_Data)  "<IMU_Data>"
  Standstill/1(standstill) -> Sensor_Select/1(standstill), Bus Creator/1  "standstill"
  Attitude_Reset/1(att_reset) -> Initial_Attitude/Enable, Bus Creator/2  "att_reset"
  Initial_Attitude/1(quat_0) -> Bus Creator/4  "quat_0"
  Bus Creator/1 -> RF_Data/1
  Attitude_Reset/2(heading_reset) -> Bus Creator/3  "heading_reset"
  Sensor_Data/1 -> Bus Selector2/1, Attitude_Reset/1(Sensor_Data), Sensor_Select/2(Sensor_Data), Initial_Attitude/1(Sensor_Data)
  Sensor_Select/1(ext_psi_enable) -> Bus Creator/5  "ext_psi_enable"
  Sensor_Select/3(mag_enable) -> Bus Creator/7  "mag_enable"
  Sensor_Select/2(gps_psi_enable) -> Bus Creator/6  "gps_psi_enable"

== system INS/Data_Fusion/Translation_Filter/CF ==
  TF_Data : Inport
  Rotation_Data : Inport  Port=2
  Bus_Constructor : Subsystem
  Horizontal_Filter : Subsystem
  Verticle_Filter : Subsystem
  Translation_Data : Outport
  wires:
  Bus_Constructor/1(Translation_Data) -> Translation_Data/1
  Verticle_Filter/1(States) -> Bus_Constructor/3(Verticle_States)
  Horizontal_Filter/1(States) -> Bus_Constructor/2(Horizontal_States)
  Rotation_Data/1 -> Verticle_Filter/2(Rotation_Data), Horizontal_Filter/2(Rotation_Data)
  TF_Data/1 -> Bus_Constructor/1(TF_Data), Verticle_Filter/1(TF_Data), Horizontal_Filter/1(TF_Data)
  Verticle_Filter/2(rf_bias) -> Bus_Constructor/4(rf_bias)

== system INS/Data_Fusion/Translation_Filter/TF_Data_PreProcess ==
  Sensor_Data : Inport
  Rotation_Data : Inport  Port=2
  Translation_Data : Inport  Port=3
  Bus Creator : BusCreator  Inputs=4
  Sensor_Process : Subsystem
  TF_Data_Post_Process : Subsystem
  Transfer_Filter_Control : Subsystem
  TF_Data : Outport
  wires:
  Sensor_Data/1 -> Sensor_Process/1(Sensor_Data)
  Translation_Data/1 -> Transfer_Filter_Control/3(Translation_Data)
  Sensor_Process/1(Sensor_Status) -> Bus Creator/1  "Sensor_Status"
  Sensor_Process/2(Sensor_Meas) -> Transfer_Filter_Control/2(Sensor_Meas), Bus Creator/2  "Sensor_Meas"
  Transfer_Filter_Control/1(TF_Control) -> Bus Creator/4  "TF_Control"
  Sensor_Process/3(Sensor_Enable) -> Transfer_Filter_Control/1(Sensor_Enable), Bus Creator/3  "Sensor_Enable"
  Rotation_Data/1 -> TF_Data_Post_Process/2(Rotation_Data), Sensor_Process/2(Rotation_Data)
  Bus Creator/1 -> TF_Data_Post_Process/1(U)
  TF_Data_Post_Process/1(Y) -> TF_Data/1

== system INS/Sensor_PreProcess/AirSpeed_Process/Calculate_IAS ==
  diff_pressure : Inport
  Abs : Abs
  AirDensity_15C : Constant  Value=1.225  OutDataTypeStr=single
  Divide : Product  Inputs=*/
  Gain : Gain  Gain=2
  Multiply : Product
  Sign : Signum
  Sqrt : Sqrt  SaturateOnIntegerOverflow=on
  IAS : Outport
  wires:
  diff_pressure/1 -> Sign/1, Abs/1
  Abs/1 -> Gain/1
  Gain/1 -> Divide/1
  AirDensity_15C/1 -> Divide/2
  Divide/1 -> Sqrt/1
  Sqrt/1 -> Multiply/2
  Sign/1 -> Multiply/1
  Multiply/1 -> IAS/1

== system INS/Sensor_PreProcess/AirSpeed_Process/Sensor_Valid ==
  Airspeed : Inport
  Bus Selector : BusSelector  OutputSignals=diff_pressure,temperature,timestamp
  Compare To Constant4 : simulink/Logic and Bit Operations/Compare To Constant  relop=<  const=timeout  OutDataTypeStr=boolean
  Constant : Constant  Value=INS_EXPORT.period  OutDataTypeStr=single
  Detect Change : simulink/Logic and Bit Operations/Detect Change  vinit=0  OutDataTypeStr=boolean
  Discrete-Time Integrator : DiscreteIntegrator  IntegratorMethod=Accumulation: Forward Euler  ExternalReset=sampled level  SampleTime=-1  OutDataTypeStr=uint32  SaturateOnIntegerOverflow=on  ICPrevOutput=DiscIntNeverNeededParam  ICPrevScaledInput=DiscIntNeverNeededParam
  Ever_Valid : Subsystem
  Interval Test1 : simulink/Logic and Bit Operations/Interval Test  IntervalClosedRight=off  uplimit=max_pressure  IntervalClosedLeft=off  lowlimit=min_pressure  OutDataTypeStr=boolean
  Interval Test2 : simulink/Logic and Bit Operations/Interval Test  IntervalClosedRight=off  uplimit=max_temp  IntervalClosedLeft=off  lowlimit=min_temp  OutDataTypeStr=boolean
  Logical Operator : Logic  AllPortsSameDT=off  OutDataTypeStr=boolean
  Logical Operator1 : Logic  Inputs=3  AllPortsSameDT=off  OutDataTypeStr=boolean
  valid : Outport
  wires:
  Interval Test1/1 -> Logical Operator/1
  Interval Test2/1 -> Logical Operator/2
  Bus Selector/2 -> Interval Test2/1  "<temperature>"
  Bus Selector/1 -> Interval Test1/1  "<diff_pressure>"
  Airspeed/1 -> Bus Selector/1
  Bus Selector/3 -> Detect Change/1  "<timestamp>"
  Discrete-Time Integrator/1 -> Compare To Constant4/1
  Constant/1 -> Discrete-Time Integrator/1
  Detect Change/1 -> Ever_Valid/1(in), Discrete-Time Integrator/2
  Logical Operator/1 -> Logical Operator1/1
  Compare To Constant4/1 -> Logical Operator1/2
  Logical Operator1/1 -> valid/1
  Ever_Valid/1(out) -> Logical Operator1/3

== system INS/Sensor_PreProcess/Baro_PreProcess/Pressure_Height ==
  pressure_Pa : Inport
  Divide : Product  Inputs=*/
  Divide1 : Product  Inputs=*/
  Gain1 : Gain  Gain=0.001
  Multiply : Product
  Power : Math  Operator=pow  SaturateOnIntegerOverflow=on
  Subtract : Sum  Inputs=+-
  T1 : Constant  Value=15+273.15  OutDataTypeStr=single
  a : Constant  Value=-6.5/1000  OutDataTypeStr=single
  aR_g : Constant  Value=-(-6.5/1000*287.05/9.80665)  OutDataTypeStr=single
  p1 : Constant  Value=101.325  OutDataTypeStr=single
  h_FL_m : Outport
  wires:
  pressure_Pa/1 -> Gain1/1
  Gain1/1 -> Divide/1  "kPp"
  Divide1/1 -> h_FL_m/1
  p1/1 -> Divide/2
  Divide/1 -> Power/1
  aR_g/1 -> Power/2
  Power/1 -> Multiply/1
  T1/1 -> Subtract/2, Multiply/2
  Multiply/1 -> Subtract/1
  Subtract/1 -> Divide1/1
  a/1 -> Divide1/2

== system INS/Sensor_PreProcess/Baro_PreProcess/Relative_Height ==
  Baro : Inport  Interpolate=off  BusOutputAsStruct=on
  data_valid : Inport  Port=2
  h_FL_m : Inport  Port=3
  Bus Selector : BusSelector  OutputSignals=timestamp
  Logical Operator : Logic  AllPortsSameDT=off  OutDataTypeStr=boolean
  Reference_Height : Subsystem
  Sampling : Subsystem
  Sum2 : Sum  Inputs=-+|
  Switch : Switch  Criteria=u2 ~= 0
  h_R_m : Outport
  baro_valid : Outport  Port=2
  wires:
  Logical Operator/1 -> baro_valid/1, Switch/2
  Bus Selector/1 -> Sampling/1(timestamp)  "<timestamp>"
  Baro/1 -> Bus Selector/1
  Sampling/1(sampling) -> Reference_Height/Enable
  Reference_Height/1(h_R_m) -> Switch/1
  Sum2/1 -> h_R_m/1
  data_valid/1 -> Logical Operator/2, Sampling/2(data_valid)
  h_FL_m/1 -> Sum2/2, Reference_Height/1(h_FL_m), Switch/3
  Switch/1 -> Sum2/1
  Sampling/2(initialized) -> Logical Operator/1

== system INS/Sensor_PreProcess/Baro_PreProcess/Sensor_Valid ==
  Baro : Inport
  Bus Selector : BusSelector  OutputSignals=pressure,temperature,timestamp
  Compare To Constant4 : simulink/Logic and Bit Operations/Compare To Constant  relop=<  const=timeout  OutDataTypeStr=boolean
  Constant : Constant  Value=INS_EXPORT.period  OutDataTypeStr=single
  Detect Change : simulink/Logic and Bit Operations/Detect Change  vinit=0  OutDataTypeStr=boolean
  Discrete-Time Integrator : DiscreteIntegrator  IntegratorMethod=Accumulation: Forward Euler  ExternalReset=sampled level  SampleTime=-1  OutDataTypeStr=uint32  SaturateOnIntegerOverflow=on  ICPrevOutput=DiscIntNeverNeededParam  ICPrevScaledInput=DiscIntNeverNeededParam
  Ever_Valid : Subsystem
  Interval Test1 : simulink/Logic and Bit Operations/Interval Test  IntervalClosedRight=off  uplimit=max_pressure  IntervalClosedLeft=off  lowlimit=min_pressure  OutDataTypeStr=boolean
  Interval Test2 : simulink/Logic and Bit Operations/Interval Test  IntervalClosedRight=off  uplimit=max_temp  IntervalClosedLeft=off  lowlimit=min_temp  OutDataTypeStr=boolean
  Logical Operator : Logic  AllPortsSameDT=off  OutDataTypeStr=boolean
  Logical Operator1 : Logic  Inputs=3  AllPortsSameDT=off  OutDataTypeStr=boolean
  valid : Outport
  wires:
  Interval Test1/1 -> Logical Operator/1
  Interval Test2/1 -> Logical Operator/2
  Bus Selector/2 -> Interval Test2/1  "<temperature>"
  Bus Selector/1 -> Interval Test1/1  "<pressure>"
  Baro/1 -> Bus Selector/1
  Bus Selector/3 -> Detect Change/1  "<timestamp>"
  Discrete-Time Integrator/1 -> Compare To Constant4/1
  Constant/1 -> Discrete-Time Integrator/1
  Detect Change/1 -> Ever_Valid/1(in), Discrete-Time Integrator/2
  Logical Operator/1 -> Logical Operator1/1
  Compare To Constant4/1 -> Logical Operator1/2
  Logical Operator1/1 -> valid/1
  Ever_Valid/1(out) -> Logical Operator1/3

== system INS/Sensor_PreProcess/ExternalPos_Process/Bus_Selector ==
  ExternalPos : Inport
  Bus Selector3 : BusSelector  OutputSignals=x,y,z,phi,theta,psi
  Gain : Gain  Gain=-1
  x : Outport
  y : Outport  Port=2
  h : Outport  Port=3
  phi : Outport  Port=4
  theta : Outport  Port=5
  psi : Outport  Port=6
  wires:
  Bus Selector3/4 -> phi/1  "<phi>"
  Bus Selector3/6 -> psi/1  "<psi>"
  Bus Selector3/5 -> theta/1  "<theta>"
  ExternalPos/1 -> Bus Selector3/1
  Bus Selector3/1 -> x/1  "<x>"
  Bus Selector3/2 -> y/1  "<y>"
  Bus Selector3/3 -> Gain/1  "<z>"
  Gain/1 -> h/1

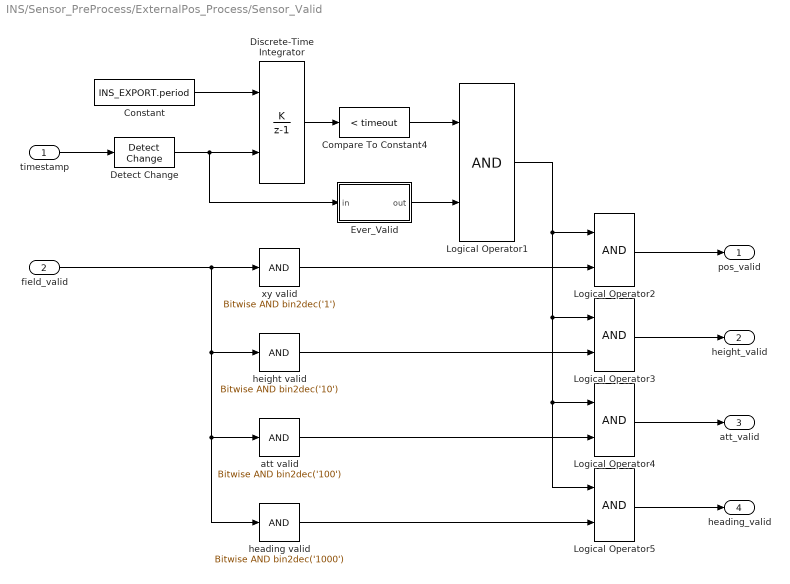
== system INS/Sensor_PreProcess/ExternalPos_Process/Sensor_Valid ==
  timestamp : Inport
  field_valid : Inport  Port=2
  Compare To Constant4 : simulink/Logic and Bit Operations/Compare To Constant  relop=<  const=timeout  OutDataTypeStr=boolean
  Constant : Constant  Value=INS_EXPORT.period  OutDataTypeStr=single
  Detect Change : simulink/Logic and Bit Operations/Detect Change  vinit=0  OutDataTypeStr=boolean
  Discrete-Time Integrator : DiscreteIntegrator  IntegratorMethod=Accumulation: Forward Euler  ExternalReset=sampled level  SampleTime=-1  OutDataTypeStr=uint32  SaturateOnIntegerOverflow=on  ICPrevOutput=DiscIntNeverNeededParam  ICPrevScaledInput=DiscIntNeverNeededParam
  Ever_Valid : Subsystem
  Logical Operator{1..5} (5 alike) : Logic  AllPortsSameDT=off  OutDataTypeStr=boolean
  att valid : simulink/Logic and Bit Operations/Bitwise Operator  logicop=AND  UseBitMask=on  BitMask=bin2dec('100')  BitMaskRealWorld=Stored Integer
  heading valid : simulink/Logic and Bit Operations/Bitwise Operator  logicop=AND  UseBitMask=on  BitMask=bin2dec('1000')  BitMaskRealWorld=Stored Integer
  height valid : simulink/Logic and Bit Operations/Bitwise Operator  logicop=AND  UseBitMask=on  BitMask=bin2dec('10')  BitMaskRealWorld=Stored Integer
  xy valid : simulink/Logic and Bit Operations/Bitwise Operator  logicop=AND  UseBitMask=on  BitMask=bin2dec('1')  BitMaskRealWorld=Stored Integer
  pos_valid : Outport
  height_valid : Outport  Port=2
  att_valid : Outport  Port=3
  heading_valid : Outport  Port=4
  wires:
  Detect Change/1 -> Ever_Valid/1(in), Discrete-Time Integrator/2
  Constant/1 -> Discrete-Time Integrator/1
  Discrete-Time Integrator/1 -> Compare To Constant4/1
  timestamp/1 -> Detect Change/1
  Compare To Constant4/1 -> Logical Operator1/1
  Ever_Valid/1(out) -> Logical Operator1/2
  field_valid/1 -> heading valid/1, att valid/1, height valid/1, xy valid/1
  Logical Operator1/1 -> Logical Operator5/1, Logical Operator4/1, Logical Operator3/1, Logical Operator2/1
  Logical Operator2/1 -> pos_valid/1
  xy valid/1 -> Logical Operator2/2
  height valid/1 -> Logical Operator3/2
  Logical Operator3/1 -> height_valid/1
  att valid/1 -> Logical Operator4/2
  heading valid/1 -> Logical Operator5/2
  Logical Operator4/1 -> att_valid/1
  Logical Operator5/1 -> heading_valid/1

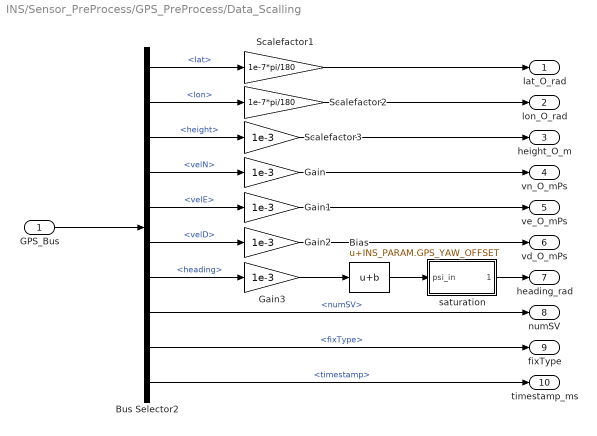
== system INS/Sensor_PreProcess/GPS_PreProcess/Data_Scalling ==
  GPS_Bus : Inport
  Bias : Bias  Bias=INS_PARAM.GPS_YAW_OFFSET
  Bus Selector2 : BusSelector  OutputSignals=lat,lon,height,velN,velE,velD,heading,numSV,fixType,timestamp
  Gain{,1..3} (4 alike) : Gain  Gain=1e-3  OutDataTypeStr=single
  Scalefactor1 : Gain  Gain=1e-7*pi/180  OutDataTypeStr=double
  Scalefactor2 : Gain  Gain=1e-7*pi/180  OutDataTypeStr=double
  Scalefactor3 : Gain  Gain=1e-3  OutDataTypeStr=double
  saturation : Subsystem
  lat_O_rad : Outport
  lon_O_rad : Outport  Port=2
  height_O_m : Outport  Port=3
  vn_O_mPs : Outport  Port=4
  ve_O_mPs : Outport  Port=5
  vd_O_mPs : Outport  Port=6
  heading_rad : Outport  Port=7
  numSV : Outport  Port=8
  fixType : Outport  Port=9
  timestamp_ms : Outport  Port=10
  wires:
  Bus Selector2/1 -> Scalefactor1/1  "<lat>"
  Bus Selector2/6 -> Gain2/1  "<velD>"
  Bus Selector2/5 -> Gain1/1  "<velE>"
  Bus Selector2/2 -> Scalefactor2/1  "<lon>"
  Scalefactor1/1 -> lat_O_rad/1
  Bus Selector2/4 -> Gain/1  "<velN>"
  Bus Selector2/3 -> Scalefactor3/1  "<height>"
  GPS_Bus/1 -> Bus Selector2/1
  Scalefactor3/1 -> height_O_m/1
  Scalefactor2/1 -> lon_O_rad/1
  Gain/1 -> vn_O_mPs/1
  Gain2/1 -> vd_O_mPs/1
  Bus Selector2/10 -> timestamp_ms/1  "<timestamp>"
  Gain1/1 -> ve_O_mPs/1
  Bus Selector2/8 -> numSV/1  "<numSV>"
  Bus Selector2/9 -> fixType/1  "<fixType>"
  Bus Selector2/7 -> Gain3/1  "<heading>"
  Gain3/1 -> Bias/1
  saturation/1(psi_rad) -> heading_rad/1
  Bias/1 -> saturation/1(psi_in)

== system INS/Sensor_PreProcess/GPS_PreProcess/Status_Quality ==
  GPS_Bus : Inport
  Bus Selector3 : BusSelector  OutputSignals=timestamp,hAcc,vAcc,sAcc,headingAcc,fixType
  Compare To Constant2 : simulink/Logic and Bit Operations/Compare To Constant  relop===  const=2  OutDataTypeStr=boolean
  GPS_Status : Subsystem
  Product{,1..3} (4 alike) : Product  Inputs=3  OutDataTypeStr=single  RndMeth=Zero
  check_timeout : Subsystem
  gps_heading_valid : Subsystem
  heading_acc : Subsystem
  horizontal_quality : Subsystem
  speed_acc : Subsystem
  vertical_quality : Subsystem
  gps_status : Outport
  spd_quality : Outport  Port=2
  hor_pos_quality : Outport  Port=3
  ver_pos_quality : Outport  Port=4
  heading_valid : Outport  Port=5
  wires:
  Bus Selector3/6 -> GPS_Status/3(fixtype)  "<fixType>"
  GPS_Bus/1 -> Bus Selector3/1
  speed_acc/1(spd_quality) -> Product2/2
  Compare To Constant2/1 -> Product1/3, Product1/1, Product/3, Product2/3, Product3/3
  Product2/1 -> spd_quality/1
  GPS_Status/1(status) -> Compare To Constant2/1, gps_status/1
  Bus Selector3/2 -> GPS_Status/2(hAcc), horizontal_quality/1(hAcc)  "<hAcc>"
  horizontal_quality/1(hor_quality) -> Product/2
  Product/1 -> gps_heading_valid/1(pos_quality), hor_pos_quality/1
  Bus Selector3/1 -> check_timeout/1(timestamp)  "<timestamp>"
  Bus Selector3/4 -> speed_acc/1(sAcc)  "<sAcc>"
  Bus Selector3/3 -> vertical_quality/1(vAcc)  "<vAcc>"
  check_timeout/1(valid) -> Product2/1, Product3/1, Product/1, GPS_Status/1(not_timeout)
  vertical_quality/1(ver_quality) -> Product1/2
  Product1/1 -> ver_pos_quality/1
  Bus Selector3/5 -> heading_acc/1(cAcc)  "<headingAcc>"
  heading_acc/1(heading_quality) -> Product3/2
  Product3/1 -> gps_heading_valid/2(yaw_quality)
  gps_heading_valid/1(valid) -> heading_valid/1

== system INS/Sensor_PreProcess/GPS_PreProcess/WGS84_Model ==
  lat_rad : Inport
  lon_rad : Inport  Port=2
  alt_m : Inport  Port=3
  Trigger : TriggerPort  VariantControl=Variant  PortDimensions=1
  Data Type Conversion : DataTypeConversion  OutDataTypeStr=double
  Data Type Conversion1 : DataTypeConversion  OutDataTypeStr=double
  LAT2FLAT Curve : FMT_Model_Lib/Transformation/LAT2FLAT Curve
      settings: SourceProductName=FMT Toolbox
  Terminator : Terminator
  constant1 : Constant  Value=-1
  lon_0_rad : Outport  InitialOutput=0
  lat_0_rad : Outport  Port=2  InitialOutput=0
  dx_dlat : Outport  Port=3  InitialOutput=1
  dy_dlon : Outport  Port=4  InitialOutput=1
  dz_dh : Outport  Port=5  InitialOutput=1
  wires:
  constant1/1 -> dz_dh/1
  alt_m/1 -> Terminator/1
  lon_rad/1 -> Data Type Conversion/1
  lat_rad/1 -> Data Type Conversion1/1
  LAT2FLAT Curve/2 -> dy_dlon/1
  LAT2FLAT Curve/1 -> dx_dlat/1
  Data Type Conversion/1 -> lon_0_rad/1
  Data Type Conversion1/1 -> lat_0_rad/1, LAT2FLAT Curve/1

== system INS/Sensor_PreProcess/IMU_PreProcess/Data_Select ==
  IMU_Bus : Inport  Interpolate=off  BusOutputAsStruct=on
  Bus Selector1 : BusSelector  OutputSignals=gyr_x,gyr_y,gyr_z,acc_x,acc_y,acc_z,timestamp
  Vector Concatenate : Concatenate  NumInputs=3  Mode=Multidimensional array
  Vector Concatenate1 : Concatenate  NumInputs=3  Mode=Multidimensional array
  gyr_B_radPs : Outport
  acc_B_mPs2 : Outport  Port=2
  timestamp_ms : Outport  Port=3
  wires:
  Bus Selector1/1 -> Vector Concatenate/1  "<gyr_x>"
  Bus Selector1/2 -> Vector Concatenate/2  "<gyr_y>"
  Bus Selector1/3 -> Vector Concatenate/3  "<gyr_z>"
  Bus Selector1/4 -> Vector Concatenate1/1  "<acc_x>"
  Bus Selector1/5 -> Vector Concatenate1/2  "<acc_y>"
  Bus Selector1/6 -> Vector Concatenate1/3  "<acc_z>"
  Bus Selector1/7 -> timestamp_ms/1  "<timestamp>"
  IMU_Bus/1 -> Bus Selector1/1
  Vector Concatenate/1 -> gyr_B_radPs/1
  Vector Concatenate1/1 -> acc_B_mPs2/1

== system INS/Sensor_PreProcess/IMU_PreProcess/Sensor_Valid ==
  gyr_B_radPs : Inport
  acc_B_mPs2 : Inport  Port=2
  timestamp_ms : Inport  Port=3
  Compare To Constant4 : simulink/Logic and Bit Operations/Compare To Constant  relop=<  const=timeout  OutDataTypeStr=boolean
  Constant : Constant  Value=INS_EXPORT.period  OutDataTypeStr=single
  Detect Change : simulink/Logic and Bit Operations/Detect Change  vinit=0  OutDataTypeStr=boolean
  Discrete-Time Integrator : DiscreteIntegrator  IntegratorMethod=Accumulation: Forward Euler  ExternalReset=sampled level  SampleTime=-1  OutDataTypeStr=uint32  SaturateOnIntegerOverflow=on  ICPrevOutput=DiscIntNeverNeededParam  ICPrevScaledInput=DiscIntNeverNeededParam
  Ever_Valid : Subsystem
  Interval Test1 : simulink/Logic and Bit Operations/Interval Test  IntervalClosedRight=off  uplimit=acc_max  IntervalClosedLeft=off  lowlimit=acc_min  OutDataTypeStr=boolean
  Interval Test3 : simulink/Logic and Bit Operations/Interval Test  IntervalClosedRight=off  uplimit=gyr_max  IntervalClosedLeft=off  lowlimit=gyr_min  OutDataTypeStr=boolean
  Logical Operator : Logic  AllPortsSameDT=off  OutDataTypeStr=boolean
  Logical Operator1 : Logic  Inputs=1  AllPortsSameDT=off  OutDataTypeStr=boolean
  Logical Operator2 : Logic  Inputs=1  AllPortsSameDT=off  OutDataTypeStr=boolean
  Logical Operator4 : Logic  Inputs=3  AllPortsSameDT=off  OutDataTypeStr=boolean
  valid : Outport
  wires:
  Logical Operator4/1 -> valid/1
  Compare To Constant4/1 -> Logical Operator4/2
  Discrete-Time Integrator/1 -> Compare To Constant4/1
  Detect Change/1 -> Ever_Valid/1(in), Discrete-Time Integrator/2
  Constant/1 -> Discrete-Time Integrator/1
  Logical Operator/1 -> Logical Operator4/1
  timestamp_ms/1 -> Detect Change/1
  Interval Test1/1 -> Logical Operator2/1
  gyr_B_radPs/1 -> Interval Test3/1
  Interval Test3/1 -> Logical Operator1/1
  Logical Operator1/1 -> Logical Operator/1
  Logical Operator2/1 -> Logical Operator/2
  acc_B_mPs2/1 -> Interval Test1/1
  Ever_Valid/1(out) -> Logical Operator4/3

== system INS/Sensor_PreProcess/MAG_PreProcess/Bus_Select ==
  MAG_Bus : Inport
  Bus Selector2 : BusSelector  OutputSignals=mag_x,mag_y,mag_z,timestamp
  Vector Concatenate2 : Concatenate  NumInputs=3  Mode=Multidimensional array
  mag_B_gauss : Outport
  timestamp_ms : Outport  Port=2
  wires:
  Bus Selector2/2 -> Vector Concatenate2/2  "<mag_y>"
  Bus Selector2/1 -> Vector Concatenate2/1  "<mag_x>"
  Vector Concatenate2/1 -> mag_B_gauss/1
  Bus Selector2/3 -> Vector Concatenate2/3  "<mag_z>"
  MAG_Bus/1 -> Bus Selector2/1
  Bus Selector2/4 -> timestamp_ms/1  "<timestamp>"
